simulink model "robot_ver2_testbench"  (R2024b)
settings: Solver=ode4  StartTime=0.0  StopTime=8  FixedStep=0.00050000000000000001  RelTol=1e-6  AbsTol=1e-8
PostLoadFcn:
  | addpath(fileparts(get_param(bdroot,'FileName')), fullfile(fileparts(get_param(bdroot,'FileName')),'src'), fullfile(fileparts(get_param(bdroot,'FileName')),'control'), fullfile(fileparts(get_param(bdroot,'FileName')),'mechanics','URDF_Assembly_Robot_ver2','meshes'));
InitFcn:
  | addpath(fileparts(get_param(bdroot,'FileName')), fullfile(fileparts(get_param(bdroot,'FileName')),'src'), fullfile(fileparts(get_param(bdroot,'FileName')),'control'), fullfile(fileparts(get_param(bdroot,'FileName')),'mechanics','URDF_Assembly_Robot_ver2','meshes'));
model workspace (MAT data in the model file):
  A6 = [0.980198019802; 0.980198019802; 0.980198019802; 0.980198019802; 0.980198019802; 0.980198019802]
  B6 = [0.00049504950495; 0.00049504950495; 0.00049504950495; 0.0049504950495; 0.0049504950495; 0.0049504950495]
  aButter = [1 -1.8226949252 0.837181651256]
  alpha = 0.118088621702
  bButter = [0.00362168151493 0.00724336302986 0.00362168151493]
  bias_est = [0; 0; 0; 0; 0; 0]
  cfg.robotID = 'robot_ver2'
  cfg.mode = 'demonstration'
  cfg.controller = 'c_sil'
  cfg.sampleTime_s = 0.002
  cfg.duration_s = 8
  cfg.gravity_m_s2 = [0 0 -9.81]
  cfg.home_deg = [0 0 -120 60 131.25 0]
  cfg.home_rad = [0 0 -2.09439510239 1.0471975512 2.29074464324 0]
  cfg.provisionalLimits_rad = [-3.14159265359  3.14159265359; -3.14159265359  3.14159265359; -3.14159265359  3.14159265359; -3.14159265359  3.14159265359; -3.14159265359  3.14159265359; -3.14159265359  3.14159265359]
  cfg.minimumLinearInverseCondition = 0.2
  cfg.minimumSelfClearance_m = 0.01
  cfg.minimumEnvironmentClearance_m = 0.01
  cfg.motionCheckStep_rad = 0.00872664625997
  cfg.startupTimeout_s = 15
  cfg.adapter.commandPort = 5006
  cfg.adapter.feedbackPort = 5007
  cfg.adapter.peer = '127.0.0.1'
  cfg.adapter.staleTimeout_s = 0.15
  cfg.adapter.maxJointStep_rad = 0.0349065850399
  cfg.upstream.controlCommit = '15aa22efc071554fe06f1e42e1007633dee15cc9'
  cfg.upstream.admittanceCommit = '589df87e0b36dfb707394ef959a6441456e408e6'
  cfg.demo.status = 'SYNTHETIC_NOT_HARDWARE'
  cfg.demo.reduction = [50 50 50 50 50 50]
  cfg.demo.encoderUnitsPerMotorRev = [32768 32768 32768 32768 32768 32768]
  cfg.demo.direction = [1 1 1 1 1 1]
  cfg.demo.zeroOffset_units = [0 0 0 0 0 0]
  cfg.demo.kp_joint_Nm_rad = [80 120 80 8 5 2]
  cfg.demo.kd_joint_Nm_s_rad = [15 20 12 0.8 0.5 0.2]
  cfg.demo.motorTorqueLimit_Nm = [4 5 4 1 0.8 0.5]
  cfg.demo.motorTorqueTimeConstant_s = 0.002
  cfg.demo.gearEfficiency = [0.9 0.9 0.9 0.9 0.9 0.9]
  cfg.demo.viscousFriction_Nm_s_rad = [0.1 0.1 0.1 0.02 0.02 0.01]
  cfg.demo.jointSpeedLimit_rad_s = [2 2 2 2 2 2]
  cfg.demo.sensor_T_flange = [1  0  0  0; 0  1  0  0; 0  0  1  0; 0  0  0  1]
  cfg.demo.virtualMass = [2 2 2 0.2 0.2 0.2]
  cfg.demo.virtualDamping = [20 20 20 2 2 2]
  cfg.demo.operatorWrench_base_tcp = [1 0 0 0 0 0]
  cfg.demo.wrenchActive_s = [1 3]
  cfg.demo.admittanceSpeedLimit = [0.05 0.05 0.05 0.15 0.15 0.15]
  cfg.demo.admittanceAccelerationLimit = [0.2 0.2 0.2 0.5 0.5 0.5]
  cfg.demo.fullJacobianMinimumSigma = 1e-06
  cfg.hardware.joints(1).motorModel = ''
  cfg.hardware.joints(1).driveModel = ''
  cfg.hardware.joints(1).gearboxModel = ''
  cfg.hardware.joints(1).ratedMotorTorque_Nm = NaN
  cfg.hardware.joints(1).peakMotorTorque_Nm = NaN
  cfg.hardware.joints(1).ratedMotorSpeed_rad_s = NaN
  cfg.hardware.joints(1).maxMotorSpeed_rad_s = NaN
  cfg.hardware.joints(1).ratedCurrent_A = NaN
  cfg.hardware.joints(1).peakCurrent_A = NaN
  cfg.hardware.joints(1).torqueConstant_Nm_A = NaN
  cfg.hardware.joints(1).resistance_Ohm = NaN
  cfg.hardware.joints(1).inductance_H = NaN
  cfg.hardware.joints(1).rotorInertia_kg_m2 = NaN
  cfg.hardware.joints(1).reduction = NaN
  cfg.hardware.joints(1).additionalReduction = NaN
  cfg.hardware.joints(1).gearEfficiency = NaN
  cfg.hardware.joints(1).gearOutputTorqueLimit_Nm = NaN
  cfg.hardware.joints(1).backlash_rad = NaN
  cfg.hardware.joints(1).torsionalStiffness_Nm_rad = NaN
  cfg.hardware.joints(1).encoderUnitsPerMotorRev = NaN
  cfg.hardware.joints(1).direction = NaN
  cfg.hardware.joints(1).zeroOffset_units = NaN
  cfg.hardware.joints(1).positionLimits_rad = [NaN NaN]
  cfg.hardware.joints(1).speedLimit_rad_s = NaN
  cfg.hardware.joints(1).accelerationLimit_rad_s2 = NaN
  cfg.hardware.joints(1).brakePresent = []
  cfg.hardware.joints(1).brakeHoldingTorque_Nm = NaN
  cfg.hardware.joints(1).brakeEngagementTime_s = NaN
  cfg.hardware.joints(1).stopBehavior = ''
  cfg.hardware.joints(1).driveControlParameters = []
  cfg.hardware.joints(1).source = ''
  cfg.hardware.joints(1).verified = 0
  cfg.hardware.joints(2).motorModel = ''
  cfg.hardware.joints(2).driveModel = ''
  cfg.hardware.joints(2).gearboxModel = ''
  cfg.hardware.joints(2).ratedMotorTorque_Nm = NaN
  cfg.hardware.joints(2).peakMotorTorque_Nm = NaN
  cfg.hardware.joints(2).ratedMotorSpeed_rad_s = NaN
  cfg.hardware.joints(2).maxMotorSpeed_rad_s = NaN
  cfg.hardware.joints(2).ratedCurrent_A = NaN
  cfg.hardware.joints(2).peakCurrent_A = NaN
  cfg.hardware.joints(2).torqueConstant_Nm_A = NaN
  cfg.hardware.joints(2).resistance_Ohm = NaN
  cfg.hardware.joints(2).inductance_H = NaN
  cfg.hardware.joints(2).rotorInertia_kg_m2 = NaN
  cfg.hardware.joints(2).reduction = NaN
  cfg.hardware.joints(2).additionalReduction = NaN
  cfg.hardware.joints(2).gearEfficiency = NaN
  cfg.hardware.joints(2).gearOutputTorqueLimit_Nm = NaN
  cfg.hardware.joints(2).backlash_rad = NaN
  cfg.hardware.joints(2).torsionalStiffness_Nm_rad = NaN
  cfg.hardware.joints(2).encoderUnitsPerMotorRev = NaN
  cfg.hardware.joints(2).direction = NaN
  cfg.hardware.joints(2).zeroOffset_units = NaN
  cfg.hardware.joints(2).positionLimits_rad = [NaN NaN]
  cfg.hardware.joints(2).speedLimit_rad_s = NaN
  cfg.hardware.joints(2).accelerationLimit_rad_s2 = NaN
  cfg.hardware.joints(2).brakePresent = []
  cfg.hardware.joints(2).brakeHoldingTorque_Nm = NaN
  cfg.hardware.joints(2).brakeEngagementTime_s = NaN
  cfg.hardware.joints(2).stopBehavior = ''
  cfg.hardware.joints(2).driveControlParameters = []
  cfg.hardware.joints(2).source = ''
  cfg.hardware.joints(2).verified = 0
  cfg.hardware.joints(3).motorModel = ''
  cfg.hardware.joints(3).driveModel = ''
  cfg.hardware.joints(3).gearboxModel = ''
  cfg.hardware.joints(3).ratedMotorTorque_Nm = NaN
  cfg.hardware.joints(3).peakMotorTorque_Nm = NaN
  cfg.hardware.joints(3).ratedMotorSpeed_rad_s = NaN
  cfg.hardware.joints(3).maxMotorSpeed_rad_s = NaN
  cfg.hardware.joints(3).ratedCurrent_A = NaN
  cfg.hardware.joints(3).peakCurrent_A = NaN
  cfg.hardware.joints(3).torqueConstant_Nm_A = NaN
  cfg.hardware.joints(3).resistance_Ohm = NaN
  cfg.hardware.joints(3).inductance_H = NaN
  cfg.hardware.joints(3).rotorInertia_kg_m2 = NaN
  cfg.hardware.joints(3).reduction = NaN
  cfg.hardware.joints(3).additionalReduction = NaN
  cfg.hardware.joints(3).gearEfficiency = NaN
  cfg.hardware.joints(3).gearOutputTorqueLimit_Nm = NaN
  cfg.hardware.joints(3).backlash_rad = NaN
  cfg.hardware.joints(3).torsionalStiffness_Nm_rad = NaN
  cfg.hardware.joints(3).encoderUnitsPerMotorRev = NaN
  cfg.hardware.joints(3).direction = NaN
  cfg.hardware.joints(3).zeroOffset_units = NaN
  cfg.hardware.joints(3).positionLimits_rad = [NaN NaN]
  cfg.hardware.joints(3).speedLimit_rad_s = NaN
  cfg.hardware.joints(3).accelerationLimit_rad_s2 = NaN
  cfg.hardware.joints(3).brakePresent = []
  cfg.hardware.joints(3).brakeHoldingTorque_Nm = NaN
  cfg.hardware.joints(3).brakeEngagementTime_s = NaN
  cfg.hardware.joints(3).stopBehavior = ''
  cfg.hardware.joints(3).driveControlParameters = []
  cfg.hardware.joints(3).source = ''
  cfg.hardware.joints(3).verified = 0
  cfg.hardware.joints(4).motorModel = ''
  cfg.hardware.joints(4).driveModel = ''
  cfg.hardware.joints(4).gearboxModel = ''
  cfg.hardware.joints(4).ratedMotorTorque_Nm = NaN
  cfg.hardware.joints(4).peakMotorTorque_Nm = NaN
  cfg.hardware.joints(4).ratedMotorSpeed_rad_s = NaN
  cfg.hardware.joints(4).maxMotorSpeed_rad_s = NaN
  cfg.hardware.joints(4).ratedCurrent_A = NaN
  cfg.hardware.joints(4).peakCurrent_A = NaN
  cfg.hardware.joints(4).torqueConstant_Nm_A = NaN
  cfg.hardware.joints(4).resistance_Ohm = NaN
  cfg.hardware.joints(4).inductance_H = NaN
  cfg.hardware.joints(4).rotorInertia_kg_m2 = NaN
  cfg.hardware.joints(4).reduction = NaN
  cfg.hardware.joints(4).additionalReduction = NaN
  cfg.hardware.joints(4).gearEfficiency = NaN
  cfg.hardware.joints(4).gearOutputTorqueLimit_Nm = NaN
  cfg.hardware.joints(4).backlash_rad = NaN
  cfg.hardware.joints(4).torsionalStiffness_Nm_rad = NaN
  cfg.hardware.joints(4).encoderUnitsPerMotorRev = NaN
  cfg.hardware.joints(4).direction = NaN
  cfg.hardware.joints(4).zeroOffset_units = NaN
  cfg.hardware.joints(4).positionLimits_rad = [NaN NaN]
  cfg.hardware.joints(4).speedLimit_rad_s = NaN
  cfg.hardware.joints(4).accelerationLimit_rad_s2 = NaN
  cfg.hardware.joints(4).brakePresent = []
  cfg.hardware.joints(4).brakeHoldingTorque_Nm = NaN
  cfg.hardware.joints(4).brakeEngagementTime_s = NaN
  cfg.hardware.joints(4).stopBehavior = ''
  cfg.hardware.joints(4).driveControlParameters = []
  cfg.hardware.joints(4).source = ''
  cfg.hardware.joints(4).verified = 0
  cfg.hardware.joints(5).motorModel = ''
  cfg.hardware.joints(5).driveModel = ''
  cfg.hardware.joints(5).gearboxModel = ''
  cfg.hardware.joints(5).ratedMotorTorque_Nm = NaN
  cfg.hardware.joints(5).peakMotorTorque_Nm = NaN
  cfg.hardware.joints(5).ratedMotorSpeed_rad_s = NaN
  cfg.hardware.joints(5).maxMotorSpeed_rad_s = NaN
  cfg.hardware.joints(5).ratedCurrent_A = NaN
  cfg.hardware.joints(5).peakCurrent_A = NaN
  cfg.hardware.joints(5).torqueConstant_Nm_A = NaN
  cfg.hardware.joints(5).resistance_Ohm = NaN
  cfg.hardware.joints(5).inductance_H = NaN
  cfg.hardware.joints(5).rotorInertia_kg_m2 = NaN
  cfg.hardware.joints(5).reduction = NaN
  cfg.hardware.joints(5).additionalReduction = NaN
  cfg.hardware.joints(5).gearEfficiency = NaN
  cfg.hardware.joints(5).gearOutputTorqueLimit_Nm = NaN
  cfg.hardware.joints(5).backlash_rad = NaN
  cfg.hardware.joints(5).torsionalStiffness_Nm_rad = NaN
  cfg.hardware.joints(5).encoderUnitsPerMotorRev = NaN
  cfg.hardware.joints(5).direction = NaN
  cfg.hardware.joints(5).zeroOffset_units = NaN
  cfg.hardware.joints(5).positionLimits_rad = [NaN NaN]
  cfg.hardware.joints(5).speedLimit_rad_s = NaN
  cfg.hardware.joints(5).accelerationLimit_rad_s2 = NaN
  cfg.hardware.joints(5).brakePresent = []
  cfg.hardware.joints(5).brakeHoldingTorque_Nm = NaN
  cfg.hardware.joints(5).brakeEngagementTime_s = NaN
  cfg.hardware.joints(5).stopBehavior = ''
  cfg.hardware.joints(5).driveControlParameters = []
  cfg.hardware.joints(5).source = ''
  cfg.hardware.joints(5).verified = 0
  cfg.hardware.joints(6).motorModel = ''
  cfg.hardware.joints(6).driveModel = ''
  cfg.hardware.joints(6).gearboxModel = ''
  cfg.hardware.joints(6).ratedMotorTorque_Nm = NaN
  cfg.hardware.joints(6).peakMotorTorque_Nm = NaN
  cfg.hardware.joints(6).ratedMotorSpeed_rad_s = NaN
  cfg.hardware.joints(6).maxMotorSpeed_rad_s = NaN
  cfg.hardware.joints(6).ratedCurrent_A = NaN
  cfg.hardware.joints(6).peakCurrent_A = NaN
  cfg.hardware.joints(6).torqueConstant_Nm_A = NaN
  cfg.hardware.joints(6).resistance_Ohm = NaN
  cfg.hardware.joints(6).inductance_H = NaN
  cfg.hardware.joints(6).rotorInertia_kg_m2 = NaN
  cfg.hardware.joints(6).reduction = NaN
  cfg.hardware.joints(6).additionalReduction = NaN
  cfg.hardware.joints(6).gearEfficiency = NaN
  cfg.hardware.joints(6).gearOutputTorqueLimit_Nm = NaN
  cfg.hardware.joints(6).backlash_rad = NaN
  cfg.hardware.joints(6).torsionalStiffness_Nm_rad = NaN
  cfg.hardware.joints(6).encoderUnitsPerMotorRev = NaN
  cfg.hardware.joints(6).direction = NaN
  cfg.hardware.joints(6).zeroOffset_units = NaN
  cfg.hardware.joints(6).positionLimits_rad = [NaN NaN]
  cfg.hardware.joints(6).speedLimit_rad_s = NaN
  cfg.hardware.joints(6).accelerationLimit_rad_s2 = NaN
  cfg.hardware.joints(6).brakePresent = []
  cfg.hardware.joints(6).brakeHoldingTorque_Nm = NaN
  cfg.hardware.joints(6).brakeEngagementTime_s = NaN
  cfg.hardware.joints(6).stopBehavior = ''
  cfg.hardware.joints(6).driveControlParameters = []
  cfg.hardware.joints(6).source = ''
  cfg.hardware.joints(6).verified = 0
  cfg.hardware.sensor.model = ''
  cfg.hardware.sensor.flange_T_sensor = [NaN  NaN  NaN  NaN; NaN  NaN  NaN  NaN; NaN  NaN  NaN  NaN; NaN  NaN  NaN  NaN]
  cfg.hardware.sensor.sensor_T_grip = [NaN  NaN  NaN  NaN; NaN  NaN  NaN  NaN; NaN  NaN  NaN  NaN; NaN  NaN  NaN  NaN]
  cfg.hardware.sensor.noiseStd = [NaN NaN NaN NaN NaN NaN]
  cfg.hardware.sensor.range = [NaN NaN NaN NaN NaN NaN]
  cfg.hardware.sensor.latency_s = NaN
  cfg.hardware.sensor.protocol = ''
  cfg.hardware.sensor.massAlreadyInCAD = []
  cfg.hardware.sensor.verified = 0
  cfg.hardware.actuatorModelValidated = 0
  cfg.hardware.massAccountingVerified = 0
  cfg.hardware.stopBehaviorValidated = 0
  cfg.hardware.source = ''
  cfg.environment(1).name = 'Floor'
  cfg.environment(1).size_m = [3 3 0.05]
  cfg.environment(1).center_m = [0 0 -0.08]
  cfg.environment(1).rpy_rad = [0 0 0]
  cfg.environment(2).name = 'Workpiece'
  cfg.environment(2).size_m = [0.3 0.3 0.1]
  cfg.environment(2).center_m = [0.85 0.65 0.35]
  cfg.environment(2).rpy_rad = [0 0 0]
  cfg.sensor.bias = [0; 0; 0; 0; 0; 0]
  cfg.sensor.noise_std = [0.08; 0.08; 0.06; 0.004; 0.004; 0.003]
  cfg.sensor.drift_per_s = [0.005; 0.003; -0.004; 0.0002; 0; 0]
  cfg.sensor.coupling = [1  0  0  0  0  0; 0  1  0  0  0  0; 0  0  1  0  0  0; 0  0  0  1  0  0; 0  0  0  0  1  0; 0  0  0  0  0  1]
  cfg.sensor.quantization_step = [0.01; 0.01; 0.01; 0.001; 0.001; 0.001]
  cfg.sensor.saturation = [100; 100; 100; 10; 10; 10]
  cfg.sensor.filterCutoff_Hz = 10
  cfg.sensor.seed = 17
  configurationSHA256 = '837b8b2e35843bef305e3cf046f537b0ec4730ac609ea7d1386ea74f346316b0'
  initialQ = [0 0 -2.09439510239 1.0471975512 2.29074464324 0]
  packagedUrdfSHA256 = '4375e6be56b72db950ac87d5631842c692121a0d0489fcb89f928996cc18049b'
undefined symbols (not defined in the file or in its folder): X, Y, Z
libraries: sm_lib x68, nesl_utility x29
(part 1 of 2)
settings Model: Creator=pc  LastModifiedBy=pc

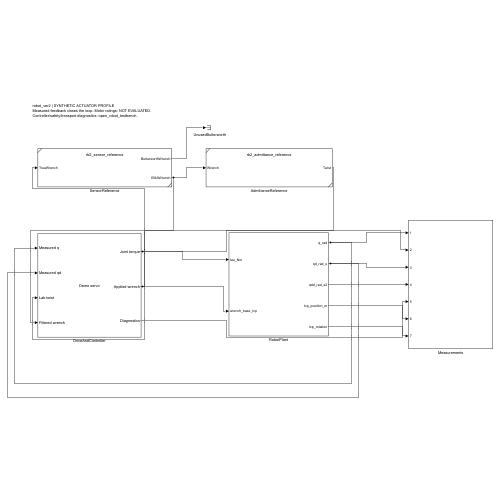
[thumbnail: Simulink's stored preview of the top-level diagram]
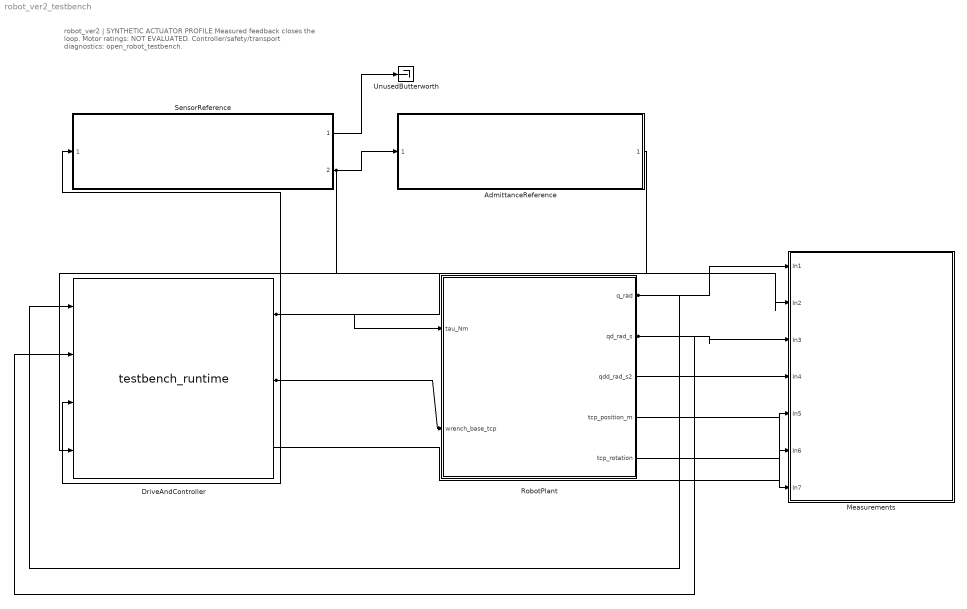
== system robot_ver2_testbench ==
  note: robot_ver2 | SYNTHETIC ACTUATOR PROFILE
      | Measured feedback closes the loop. Motor ratings: NOT EVALUATED.
      | Controller/safety/transport diagnostics: open_robot_testbench.
  AdmittanceReference : Subsystem  ReferencedSubsystem=rb2_admittance_reference
  DriveAndController : M-S-Function  FunctionName=testbench_runtime
      mask Display:
      | disp('Demo servo');
      | port_label('input',1,'Measured q');port_label('input',2,'Measured qd');
      | port_label('input',3,'Lab twist');port_label('input',4,'Filtered wrench');
      | port_label('output',1,'Joint torque');port_label('output',2,'Applied wrench');
      | port_label('output',3,'Diagnostics');
  Measurements : Subsystem
  RobotPlant : Subsystem
  SensorReference : Subsystem  ReferencedSubsystem=rb2_sensor_reference
  UnusedButterworth : Terminator
  wires:
  SensorReference/2 -> AdmittanceReference/1, DriveAndController/4
  RobotPlant/1(q_rad) -> DriveAndController/1, Measurements/1(In1)
  RobotPlant/2(qd_rad_s) -> DriveAndController/2, Measurements/3(In3)
  AdmittanceReference/1 -> DriveAndController/3
  DriveAndController/1 -> Measurements/2(In2), RobotPlant/1(tau_Nm)
  RobotPlant/3(qdd_rad_s2) -> Measurements/4(In4)
  DriveAndController/3 -> Measurements/5(In5)
  RobotPlant/4(tcp_position_m) -> Measurements/6(In6)
  RobotPlant/5(tcp_rotation) -> Measurements/7(In7)
  DriveAndController/2 -> RobotPlant/2(wrench_base_tcp), SensorReference/1
  SensorReference/1 -> UnusedButterworth/1

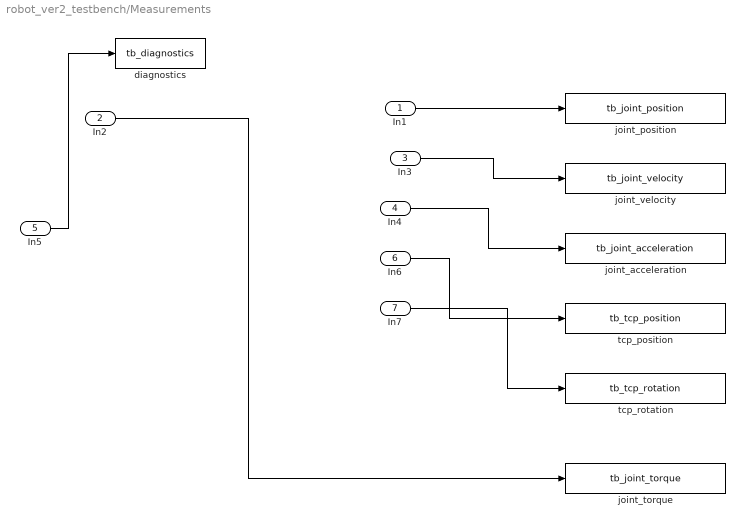
== system robot_ver2_testbench/Measurements ==
  In1 : Inport
  In2 : Inport  Port=2
  In3 : Inport  Port=3
  In4 : Inport  Port=4
  In5 : Inport  Port=5
  In6 : Inport  Port=6
  In7 : Inport  Port=7
  diagnostics : ToWorkspace  VariableName=tb_diagnostics  SaveFormat=Timeseries  SampleTime=-1
  joint_acceleration : ToWorkspace  VariableName=tb_joint_acceleration  SaveFormat=Timeseries  SampleTime=-1
  joint_position : ToWorkspace  VariableName=tb_joint_position  SaveFormat=Timeseries  SampleTime=-1
  joint_torque : ToWorkspace  VariableName=tb_joint_torque  SaveFormat=Timeseries  SampleTime=-1
  joint_velocity : ToWorkspace  VariableName=tb_joint_velocity  SaveFormat=Timeseries  SampleTime=-1
  tcp_position : ToWorkspace  VariableName=tb_tcp_position  SaveFormat=Timeseries  SampleTime=-1
  tcp_rotation : ToWorkspace  VariableName=tb_tcp_rotation  SaveFormat=Timeseries  SampleTime=-1
  wires:
  In7/1 -> tcp_rotation/1
  In3/1 -> joint_velocity/1
  In5/1 -> diagnostics/1
  In6/1 -> tcp_position/1
  In2/1 -> joint_torque/1
  In4/1 -> joint_acceleration/1
  In1/1 -> joint_position/1

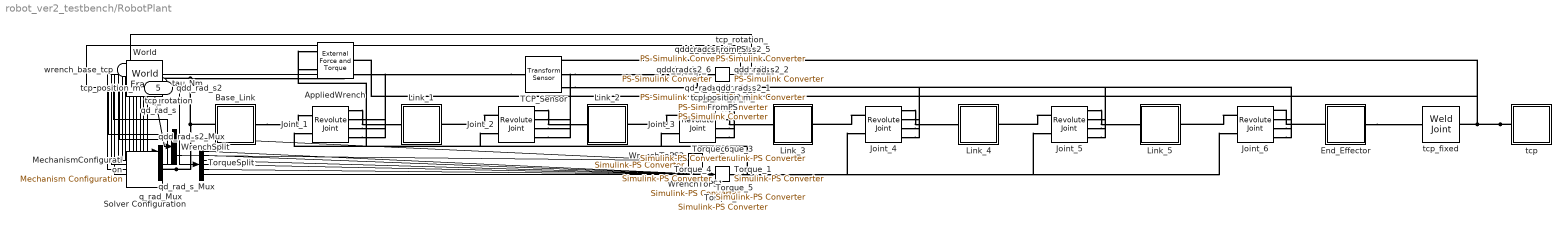
== system robot_ver2_testbench/RobotPlant ==
  tau_Nm : Inport  PortDimensions=6
  wrench_base_tcp : Inport  Port=2  PortDimensions=6
  AppliedWrench : sm_lib/Forces and Torques/External Force and Torque  EnableForceX=off  EnableForceY=off  EnableForceZ=off  EnableForce=on  ForceResolutionFrame=World  EnableTorqueX=off  EnableTorqueY=off  EnableTorqueZ=off  EnableTorque=on  TorqueResolutionFrame=World
  Base_Link : Subsystem
  End_Effector : Subsystem
  Joint_1 : sm_lib/Joints/Revolute Joint  JointMode=Normal  CompositeWrenchDir=FollowerOnBase  CompositeWrenchFrame=BaseFrame  SenseConstraintForce=off  SenseConstraintTorque=off  SenseTotalForce=off  SenseTotalTorque=off  PositionTargetSpecify=on  PositionTargetPriority=High  PositionTargetValue=initialQ(1)  PositionTargetValueUnits=rad  VelocityTargetSpecify=on  VelocityTargetPriority=High  VelocityTargetValue=0  VelocityTargetValueUnits=rad/s  EquilibriumPosition=0  EquilibriumPositionUnits=deg  SpringStiffness=0  SpringStiffnessUnits=N*m/deg  DampingCoefficient=0  DampingCoefficientUnits=kg*m^2/(rad*s)  LowerLimitSpecify=on  LowerLimitBound=-3.141592653589793  LowerLimitBoundUnits=rad  LowerLimitStiffness=1e4  LowerLimitStiffnessUnits=N*m/deg  LowerLimitDamping=10  LowerLimitDampingUnits=N*m/(deg/s)  LowerLimitTransitionRegionWidth=0.1  LowerLimitTransitionRegionWidthUnits=deg  UpperLimitSpecify=on  UpperLimitBound=3.141592653589793  UpperLimitBoundUnits=rad  UpperLimitStiffness=1e4  UpperLimitStiffnessUnits=N*m/deg  UpperLimitDamping=10  UpperLimitDampingUnits=N*m/(deg/s)  UpperLimitTransitionRegionWidth=0.1  UpperLimitTransitionRegionWidthUnits=deg  TorqueActuationMode=InputTorque  MotionActuationMode=ComputedMotion  SensePosition=on  SenseVelocity=on  SenseAcceleration=on  SenseTorqueForce=off  SenseLowerLimitTorqueForce=off  SenseUpperLimitTorqueForce=off
  Joint_2 : sm_lib/Joints/Revolute Joint  JointMode=Normal  CompositeWrenchDir=FollowerOnBase  CompositeWrenchFrame=BaseFrame  SenseConstraintForce=off  SenseConstraintTorque=off  SenseTotalForce=off  SenseTotalTorque=off  PositionTargetSpecify=on  PositionTargetPriority=High  PositionTargetValue=initialQ(2)  PositionTargetValueUnits=rad  VelocityTargetSpecify=on  VelocityTargetPriority=High  VelocityTargetValue=0  VelocityTargetValueUnits=rad/s  EquilibriumPosition=0  EquilibriumPositionUnits=deg  SpringStiffness=0  SpringStiffnessUnits=N*m/deg  DampingCoefficient=0  DampingCoefficientUnits=kg*m^2/(rad*s)  LowerLimitSpecify=on  LowerLimitBound=-3.141592653589793  LowerLimitBoundUnits=rad  LowerLimitStiffness=1e4  LowerLimitStiffnessUnits=N*m/deg  LowerLimitDamping=10  LowerLimitDampingUnits=N*m/(deg/s)  LowerLimitTransitionRegionWidth=0.1  LowerLimitTransitionRegionWidthUnits=deg  UpperLimitSpecify=on  UpperLimitBound=3.141592653589793  UpperLimitBoundUnits=rad  UpperLimitStiffness=1e4  UpperLimitStiffnessUnits=N*m/deg  UpperLimitDamping=10  UpperLimitDampingUnits=N*m/(deg/s)  UpperLimitTransitionRegionWidth=0.1  UpperLimitTransitionRegionWidthUnits=deg  TorqueActuationMode=InputTorque  MotionActuationMode=ComputedMotion  SensePosition=on  SenseVelocity=on  SenseAcceleration=on  SenseTorqueForce=off  SenseLowerLimitTorqueForce=off  SenseUpperLimitTorqueForce=off
  Joint_3 : sm_lib/Joints/Revolute Joint  JointMode=Normal  CompositeWrenchDir=FollowerOnBase  CompositeWrenchFrame=BaseFrame  SenseConstraintForce=off  SenseConstraintTorque=off  SenseTotalForce=off  SenseTotalTorque=off  PositionTargetSpecify=on  PositionTargetPriority=High  PositionTargetValue=initialQ(3)  PositionTargetValueUnits=rad  VelocityTargetSpecify=on  VelocityTargetPriority=High  VelocityTargetValue=0  VelocityTargetValueUnits=rad/s  EquilibriumPosition=0  EquilibriumPositionUnits=deg  SpringStiffness=0  SpringStiffnessUnits=N*m/deg  DampingCoefficient=0  DampingCoefficientUnits=kg*m^2/(rad*s)  LowerLimitSpecify=on  LowerLimitBound=-3.141592653589793  LowerLimitBoundUnits=rad  LowerLimitStiffness=1e4  LowerLimitStiffnessUnits=N*m/deg  LowerLimitDamping=10  LowerLimitDampingUnits=N*m/(deg/s)  LowerLimitTransitionRegionWidth=0.1  LowerLimitTransitionRegionWidthUnits=deg  UpperLimitSpecify=on  UpperLimitBound=3.141592653589793  UpperLimitBoundUnits=rad  UpperLimitStiffness=1e4  UpperLimitStiffnessUnits=N*m/deg  UpperLimitDamping=10  UpperLimitDampingUnits=N*m/(deg/s)  UpperLimitTransitionRegionWidth=0.1  UpperLimitTransitionRegionWidthUnits=deg  TorqueActuationMode=InputTorque  MotionActuationMode=ComputedMotion  SensePosition=on  SenseVelocity=on  SenseAcceleration=on  SenseTorqueForce=off  SenseLowerLimitTorqueForce=off  SenseUpperLimitTorqueForce=off
  Joint_4 : sm_lib/Joints/Revolute Joint  JointMode=Normal  CompositeWrenchDir=FollowerOnBase  CompositeWrenchFrame=BaseFrame  SenseConstraintForce=off  SenseConstraintTorque=off  SenseTotalForce=off  SenseTotalTorque=off  PositionTargetSpecify=on  PositionTargetPriority=High  PositionTargetValue=initialQ(4)  PositionTargetValueUnits=rad  VelocityTargetSpecify=on  VelocityTargetPriority=High  VelocityTargetValue=0  VelocityTargetValueUnits=rad/s  EquilibriumPosition=0  EquilibriumPositionUnits=deg  SpringStiffness=0  SpringStiffnessUnits=N*m/deg  DampingCoefficient=0  DampingCoefficientUnits=kg*m^2/(rad*s)  LowerLimitSpecify=on  LowerLimitBound=-3.141592653589793  LowerLimitBoundUnits=rad  LowerLimitStiffness=1e4  LowerLimitStiffnessUnits=N*m/deg  LowerLimitDamping=10  LowerLimitDampingUnits=N*m/(deg/s)  LowerLimitTransitionRegionWidth=0.1  LowerLimitTransitionRegionWidthUnits=deg  UpperLimitSpecify=on  UpperLimitBound=3.141592653589793  UpperLimitBoundUnits=rad  UpperLimitStiffness=1e4  UpperLimitStiffnessUnits=N*m/deg  UpperLimitDamping=10  UpperLimitDampingUnits=N*m/(deg/s)  UpperLimitTransitionRegionWidth=0.1  UpperLimitTransitionRegionWidthUnits=deg  TorqueActuationMode=InputTorque  MotionActuationMode=ComputedMotion  SensePosition=on  SenseVelocity=on  SenseAcceleration=on  SenseTorqueForce=off  SenseLowerLimitTorqueForce=off  SenseUpperLimitTorqueForce=off
  Joint_5 : sm_lib/Joints/Revolute Joint  JointMode=Normal  CompositeWrenchDir=FollowerOnBase  CompositeWrenchFrame=BaseFrame  SenseConstraintForce=off  SenseConstraintTorque=off  SenseTotalForce=off  SenseTotalTorque=off  PositionTargetSpecify=on  PositionTargetPriority=High  PositionTargetValue=initialQ(5)  PositionTargetValueUnits=rad  VelocityTargetSpecify=on  VelocityTargetPriority=High  VelocityTargetValue=0  VelocityTargetValueUnits=rad/s  EquilibriumPosition=0  EquilibriumPositionUnits=deg  SpringStiffness=0  SpringStiffnessUnits=N*m/deg  DampingCoefficient=0  DampingCoefficientUnits=kg*m^2/(rad*s)  LowerLimitSpecify=on  LowerLimitBound=-3.141592653589793  LowerLimitBoundUnits=rad  LowerLimitStiffness=1e4  LowerLimitStiffnessUnits=N*m/deg  LowerLimitDamping=10  LowerLimitDampingUnits=N*m/(deg/s)  LowerLimitTransitionRegionWidth=0.1  LowerLimitTransitionRegionWidthUnits=deg  UpperLimitSpecify=on  UpperLimitBound=3.141592653589793  UpperLimitBoundUnits=rad  UpperLimitStiffness=1e4  UpperLimitStiffnessUnits=N*m/deg  UpperLimitDamping=10  UpperLimitDampingUnits=N*m/(deg/s)  UpperLimitTransitionRegionWidth=0.1  UpperLimitTransitionRegionWidthUnits=deg  TorqueActuationMode=InputTorque  MotionActuationMode=ComputedMotion  SensePosition=on  SenseVelocity=on  SenseAcceleration=on  SenseTorqueForce=off  SenseLowerLimitTorqueForce=off  SenseUpperLimitTorqueForce=off
  Joint_6 : sm_lib/Joints/Revolute Joint  JointMode=Normal  CompositeWrenchDir=FollowerOnBase  CompositeWrenchFrame=BaseFrame  SenseConstraintForce=off  SenseConstraintTorque=off  SenseTotalForce=off  SenseTotalTorque=off  PositionTargetSpecify=on  PositionTargetPriority=High  PositionTargetValue=initialQ(6)  PositionTargetValueUnits=rad  VelocityTargetSpecify=on  VelocityTargetPriority=High  VelocityTargetValue=0  VelocityTargetValueUnits=rad/s  EquilibriumPosition=0  EquilibriumPositionUnits=deg  SpringStiffness=0  SpringStiffnessUnits=N*m/deg  DampingCoefficient=0  DampingCoefficientUnits=kg*m^2/(rad*s)  LowerLimitSpecify=on  LowerLimitBound=-3.141592653589793  LowerLimitBoundUnits=rad  LowerLimitStiffness=1e4  LowerLimitStiffnessUnits=N*m/deg  LowerLimitDamping=10  LowerLimitDampingUnits=N*m/(deg/s)  LowerLimitTransitionRegionWidth=0.1  LowerLimitTransitionRegionWidthUnits=deg  UpperLimitSpecify=on  UpperLimitBound=3.141592653589793  UpperLimitBoundUnits=rad  UpperLimitStiffness=1e4  UpperLimitStiffnessUnits=N*m/deg  UpperLimitDamping=10  UpperLimitDampingUnits=N*m/(deg/s)  UpperLimitTransitionRegionWidth=0.1  UpperLimitTransitionRegionWidthUnits=deg  TorqueActuationMode=InputTorque  MotionActuationMode=ComputedMotion  SensePosition=on  SenseVelocity=on  SenseAcceleration=on  SenseTorqueForce=off  SenseLowerLimitTorqueForce=off  SenseUpperLimitTorqueForce=off
  Link_1 : Subsystem
  Link_2 : Subsystem
  Link_3 : Subsystem
  Link_4 : Subsystem
  Link_5 : Subsystem
  MechanismConfiguration : sm_lib/Utilities/Mechanism Configuration  UniformGravity=Constant  GravityVector=[0 0 -9.8100000000000005]  GravityVectorUnits=m/s^2  LinearizationDelta=0.001  JointModeTransitionNonlinearIterations=2
  Solver Configuration : nesl_utility/Solver Configuration  PhysicalDomain=network_engine_domain  SubClassName=solver  LeftPortType=input  RightPortType=generic  Tones=[]  Harmonics=[]  SimulateNoise=off  Profile=off  UseLocalSampling=off  EnableSwitchedLinearOptims=on  FrequencyDomain=off  UseCCode=off  RelTol=0.001  AbsTol=0.001  MinStep=1e-09  ToWorkspace=off  RevertToSquareIcSolve=off  NumHomotopyIterations=100  PhasorMode=off  PhasorModeNumHarmonics=1  ConsistencySolver=NEWTON_XTOL_AFTER_FTOL  IndexReductionMethod=DerivativeReplacement  DoDC=off  ResidualTolerance=1e-09  ConsistencyTolSource=GLOBAL  ConsistencyAbsTol=0.001  ConsistencyRelTol=0.001  ConsistencyTolFactor=0.001  UseLocalSolver=off  LocalSolverChoice=NE_BACKWARD_EULER_ADVANCER  ResolveIndetEquations=on  FunctionEvalNumThread=1  LocalSolverSampleTime=0.001  DoFixedCost=off  MaxNonlinIter=3  MaxModeIter=2  ComputeImpulses=off  ImpulseIterations=2  LinearAlgebra=auto  LinearAlgebraNumThread=0  EquationFormulation=NE_TIME_EF  DelaysMemoryBudget=1024  AutomaticFiltering=on  FilteringTimeConstant=0.001  PartitionStorageMethod=AS_NEEDED  PartitionMemoryBudget=1024  PartitionMethod=ROBUST  MultibodyUseLocalSolver=off  MultibodyLocalSolverChoice=ODE1  MultibodyLocalSolverSampleTime=0.001
  TCP_Sensor : sm_lib/Frames and Transforms/Transform Sensor  MeasurementFrame=World  RotationSequence=XYX  SenseAngle=off  SenseAxis=off  SenseQ=off  SenseR=on  SenseRotationSequence=off  SenseOmegaX=off  SenseOmegaY=off  SenseOmegaZ=off  SenseOmega=off  SenseQDot=off  SenseRDot=off  SenseRotationSequenceDot=off  SenseAlphaX=off  SenseAlphaY=off  SenseAlphaZ=off  SenseAlpha=off  SenseQDDot=off  SenseRDDot=off  SenseX=off  SenseY=off  SenseZ=off  SenseXYZ=on  SenseRad=off  SenseAzim=off  SenseDist=off  SenseInc=off  SenseXDot=off  SenseYDot=off  SenseZDot=off  SenseXYZDot=off  SenseRadDot=off  SenseAzimDot=off  SenseDistDot=off  SenseIncDot=off  SenseXDDot=off  SenseYDDot=off  SenseZDDot=off  SenseXYZDDot=off  SenseRadDDot=off  SenseAzimDDot=off  SenseDistDDot=off  SenseIncDDot=off
  TorqueSplit : Demux  Outputs=6
  Torque_{1..6} (6 alike) : nesl_utility/Simulink-PS Converter  PhysicalDomain=network_engine_domain  SubClassName=ps_input  LeftPortType=input  RightPortType=output  PseudoPeriodic=off  Frequencies=[]  NoiseDistribution=none  NoiseParameters=[]  Unit=N*m  AffineConversion=off  FilteringAndDerivatives=provide  SimscapeFilterOrder=1  InputFilterTimeConstant=0.001  UdotUserProvided=0
  World : sm_lib/Frames and Transforms/World Frame
  WrenchSplit : Demux  Outputs=[3 3]
  WrenchToPS1 : nesl_utility/Simulink-PS Converter  PhysicalDomain=network_engine_domain  SubClassName=ps_input  LeftPortType=input  RightPortType=output  PseudoPeriodic=off  Frequencies=[]  NoiseDistribution=none  NoiseParameters=[]  Unit=N  AffineConversion=off  FilteringAndDerivatives=provide  SimscapeFilterOrder=1  InputFilterTimeConstant=0.001  UdotUserProvided=0
  WrenchToPS2 : nesl_utility/Simulink-PS Converter  PhysicalDomain=network_engine_domain  SubClassName=ps_input  LeftPortType=input  RightPortType=output  PseudoPeriodic=off  Frequencies=[]  NoiseDistribution=none  NoiseParameters=[]  Unit=N*m  AffineConversion=off  FilteringAndDerivatives=provide  SimscapeFilterOrder=1  InputFilterTimeConstant=0.001  UdotUserProvided=0
  q_rad_{1..6} (6 alike) : nesl_utility/PS-Simulink Converter  PhysicalDomain=network_engine_domain  SubClassName=ps_output  LeftPortType=input  RightPortType=output  PseudoPeriodic=off  Frequencies=[]  VectorFormat=inherit  Unit=rad  AffineConversion=off
  q_rad_Mux : Mux  Inputs=6
  qd_rad_s_{1..6} (6 alike) : nesl_utility/PS-Simulink Converter  PhysicalDomain=network_engine_domain  SubClassName=ps_output  LeftPortType=input  RightPortType=output  PseudoPeriodic=off  Frequencies=[]  VectorFormat=inherit  Unit=rad/s  AffineConversion=off
  qd_rad_s_Mux : Mux  Inputs=6
  qdd_rad_s2_{1..6} (6 alike) : nesl_utility/PS-Simulink Converter  PhysicalDomain=network_engine_domain  SubClassName=ps_output  LeftPortType=input  RightPortType=output  PseudoPeriodic=off  Frequencies=[]  VectorFormat=inherit  Unit=rad/s^2  AffineConversion=off
  qdd_rad_s2_Mux : Mux  Inputs=6
  tcp : Subsystem
  tcp_fixed : sm_lib/Joints/Weld Joint  JointMode=Normal  CompositeWrenchDir=FollowerOnBase  CompositeWrenchFrame=BaseFrame  SenseConstraintForce=off  SenseConstraintTorque=off  SenseTotalForce=off  SenseTotalTorque=off
  tcp_position_m_FromPS : nesl_utility/PS-Simulink Converter  PhysicalDomain=network_engine_domain  SubClassName=ps_output  LeftPortType=input  RightPortType=output  PseudoPeriodic=off  Frequencies=[]  VectorFormat=inherit  Unit=m  AffineConversion=off
  tcp_rotation_FromPS : nesl_utility/PS-Simulink Converter  PhysicalDomain=network_engine_domain  SubClassName=ps_output  LeftPortType=input  RightPortType=output  PseudoPeriodic=off  Frequencies=[]  VectorFormat=inherit  Unit=1  AffineConversion=off
  q_rad : Outport
  qd_rad_s : Outport  Port=2
  qdd_rad_s2 : Outport  Port=3
  tcp_position_m : Outport  Port=4
  tcp_rotation : Outport  Port=5
  wires:
  qdd_rad_s2_2/1 -> qdd_rad_s2_Mux/2
  q_rad_2/1 -> q_rad_Mux/2
  qd_rad_s_2/1 -> qd_rad_s_Mux/2
  TorqueSplit/2 -> Torque_2/1
  qd_rad_s_Mux/1 -> qd_rad_s/1
  TorqueSplit/5 -> Torque_5/1
  qd_rad_s_5/1 -> qd_rad_s_Mux/5
  qdd_rad_s2_6/1 -> qdd_rad_s2_Mux/6
  TorqueSplit/1 -> Torque_1/1
  TorqueSplit/6 -> Torque_6/1
  qdd_rad_s2_4/1 -> qdd_rad_s2_Mux/4
  qdd_rad_s2_3/1 -> qdd_rad_s2_Mux/3
  q_rad_3/1 -> q_rad_Mux/3
  qd_rad_s_4/1 -> qd_rad_s_Mux/4
  q_rad_6/1 -> q_rad_Mux/6
  tcp_position_m_FromPS/1 -> tcp_position_m/1
  qdd_rad_s2_Mux/1 -> qdd_rad_s2/1
  q_rad_4/1 -> q_rad_Mux/4
  qdd_rad_s2_5/1 -> qdd_rad_s2_Mux/5
  qd_rad_s_3/1 -> qd_rad_s_Mux/3
  qd_rad_s_1/1 -> qd_rad_s_Mux/1
  tcp_rotation_FromPS/1 -> tcp_rotation/1
  qdd_rad_s2_1/1 -> qdd_rad_s2_Mux/1
  q_rad_5/1 -> q_rad_Mux/5
  q_rad_Mux/1 -> q_rad/1
  tau_Nm/1 -> TorqueSplit/1
  qd_rad_s_6/1 -> qd_rad_s_Mux/6
  q_rad_1/1 -> q_rad_Mux/1
  TorqueSplit/3 -> Torque_3/1
  TorqueSplit/4 -> Torque_4/1
  wrench_base_tcp/1 -> WrenchSplit/1
  WrenchSplit/1 -> WrenchToPS1/1
  WrenchSplit/2 -> WrenchToPS2/1
  connections:
  Joint_2/RConn2 -- q_rad_2/LConn1
  Torque_2/RConn1 -- Joint_2/LConn2
  Joint_1/RConn4 -- qdd_rad_s2_1/LConn1
  Joint_2/RConn3 -- qd_rad_s_2/LConn1
  Joint_2/RConn4 -- qdd_rad_s2_2/LConn1
  TCP_Sensor/RConn3 -- tcp_position_m_FromPS/LConn1
  Joint_5/RConn3 -- qd_rad_s_5/LConn1
  Torque_1/RConn1 -- Joint_1/LConn2
  Joint_4/RConn2 -- q_rad_4/LConn1
  Joint_3/RConn3 -- qd_rad_s_3/LConn1
  Joint_6/RConn4 -- qdd_rad_s2_6/LConn1
  Joint_3/RConn2 -- q_rad_3/LConn1
  Torque_3/RConn1 -- Joint_3/LConn2
  Joint_4/RConn4 -- qdd_rad_s2_4/LConn1
  Torque_4/RConn1 -- Joint_4/LConn2
  Joint_1/RConn3 -- qd_rad_s_1/LConn1
  Joint_1/RConn1 -- Link_1/LConn1
  Joint_4/RConn3 -- qd_rad_s_4/LConn1
  End_Effector/LConn1 -- Joint_6/RConn1
  Torque_6/RConn1 -- Joint_6/LConn2
  Base_Link/RConn1 -- Joint_1/LConn1
  End_Effector/RConn1 -- tcp_fixed/LConn1
  Joint_3/LConn1 -- Link_2/RConn1
  Joint_5/RConn4 -- qdd_rad_s2_5/LConn1
  Joint_3/RConn1 -- Link_3/LConn1
  Joint_5/RConn2 -- q_rad_5/LConn1
  Joint_2/RConn1 -- Link_2/LConn1
  Torque_5/RConn1 -- Joint_5/LConn2
  Joint_6/RConn3 -- qd_rad_s_6/LConn1
  Joint_4/LConn1 -- Link_3/RConn1
  Joint_4/RConn1 -- Link_4/LConn1
  Joint_5/RConn1 -- Link_5/LConn1
  Joint_5/LConn1 -- Link_4/RConn1
  Joint_1/RConn2 -- q_rad_1/LConn1
  Joint_6/LConn1 -- Link_5/RConn1
  TCP_Sensor/RConn2 -- tcp_rotation_FromPS/LConn1
  Joint_6/RConn2 -- q_rad_6/LConn1
  TCP_Sensor/LConn1 -- World/RConn1 -- Solver Configuration/RConn1 -- MechanismConfiguration/RConn1 -- Base_Link/LConn1
  TCP_Sensor/RConn1 -- tcp/LConn1 -- AppliedWrench/RConn1 -- tcp_fixed/RConn1
  Joint_3/RConn4 -- qdd_rad_s2_3/LConn1
  Joint_2/LConn1 -- Link_1/RConn1
  WrenchToPS1/RConn1 -- AppliedWrench/LConn1
  WrenchToPS2/RConn1 -- AppliedWrench/LConn2

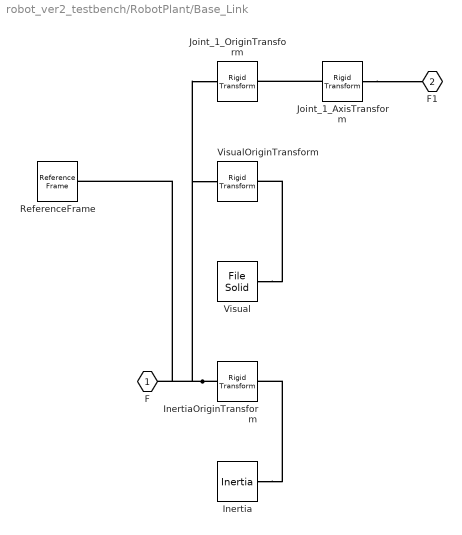
== system robot_ver2_testbench/RobotPlant/Base_Link ==
  Inertia : sm_lib/Body Elements/Inertia  InertiaType=Custom  Mass=4.45952773181733  MassUnits=kg  CenterOfMass=[0, 0, 0]  CenterOfMassUnits=m  MomentsOfInertia=[0.0365014937398595, 0.0365014937398595, 0.0432728026009368]  MomentsOfInertiaUnits=kg*m^2  ProductsOfInertia=[-1.63931612712631e-18, 3.25877544074145e-19, -1.11173074327127e-18]  ProductsOfInertiaUnits=kg*m^2  GraphicType=None  MarkerShape=Inertia  MarkerSize=20  GraphicVisPropType=SimpleVisualProperties  GraphicDiffuseColor=[0.5 0.5 0.5]  GraphicOpacity=1  GraphicSpecularColor=[0.5 0.5 0.5 1.0]  GraphicAmbientColor=[0.15 0.15 0.15 1.0]  GraphicEmissiveColor=[0.0 0.0 0.0 1.0]  GraphicShininess=75
  InertiaOriginTransform : sm_lib/Frames and Transforms/Rigid Transform  RotationMethod=RotationSequence  FollAlignAxisA=+X  BaseAlignAxisA=+Y  FollAlignAxisB=+Y  BaseAlignAxisB=+Z  RotationStandardAxis=+Z  RotationAngle=0  RotationAngleUnits=deg  RotationArbitraryAxis=[0 0 1]  RotationSequenceAxes=BaseAxes  RotationSequence=XYZ  RotationSequenceAngles=[0, 0, 0]  RotationSequenceAnglesUnits=rad  RotationMatrix=[1 0 0;0 1 0;0 0 1]  Quaternion=[1 0 0 0]  TranslationMethod=Cartesian  TranslationCartesianOffset=[7.32447693854411e-18, -1.19067266926414e-17, 0.1]  TranslationCartesianOffsetUnits=m  TranslationStandardAxis=+Z  TranslationStandardOffset=0  TranslationStandardOffsetUnits=m  TranslationROffset=0  TranslationROffsetUnits=m  TranslationThetaOffset=0  TranslationThetaOffsetUnits=deg  TranslationZOffset=0  TranslationZOffsetUnits=m
  Joint_1_AxisTransform : sm_lib/Frames and Transforms/Rigid Transform  RotationMethod=ArbitraryAxis  FollAlignAxisA=+X  BaseAlignAxisA=+Y  FollAlignAxisB=+Y  BaseAlignAxisB=+Z  RotationStandardAxis=+Z  RotationAngle=3.141592653589793  RotationAngleUnits=rad  RotationArbitraryAxis=[1, 0, 0]  RotationSequenceAxes=FollowerAxes  RotationSequence=XYX  RotationSequenceAngles=[0 0 0]  RotationSequenceAnglesUnits=deg  RotationMatrix=[1 0 0;0 1 0;0 0 1]  Quaternion=[1 0 0 0]  TranslationMethod=Cartesian  TranslationCartesianOffset=[0, 0, 0]  TranslationCartesianOffsetUnits=m  TranslationStandardAxis=+Z  TranslationStandardOffset=0  TranslationStandardOffsetUnits=m  TranslationROffset=0  TranslationROffsetUnits=m  TranslationThetaOffset=0  TranslationThetaOffsetUnits=deg  TranslationZOffset=0  TranslationZOffsetUnits=m
  Joint_1_OriginTransform : sm_lib/Frames and Transforms/Rigid Transform  RotationMethod=RotationSequence  FollAlignAxisA=+X  BaseAlignAxisA=+Y  FollAlignAxisB=+Y  BaseAlignAxisB=+Z  RotationStandardAxis=+Z  RotationAngle=0  RotationAngleUnits=deg  RotationArbitraryAxis=[0 0 1]  RotationSequenceAxes=BaseAxes  RotationSequence=XYZ  RotationSequenceAngles=[0, 0, 0]  RotationSequenceAnglesUnits=rad  RotationMatrix=[1 0 0;0 1 0;0 0 1]  Quaternion=[1 0 0 0]  TranslationMethod=Cartesian  TranslationCartesianOffset=[0, 0, 0.2]  TranslationCartesianOffsetUnits=m  TranslationStandardAxis=+Z  TranslationStandardOffset=0  TranslationStandardOffsetUnits=m  TranslationROffset=0  TranslationROffsetUnits=m  TranslationThetaOffset=0  TranslationThetaOffsetUnits=deg  TranslationZOffset=0  TranslationZOffsetUnits=m
  ReferenceFrame : sm_lib/Frames and Transforms/Reference Frame
  Visual : sm_lib/Body Elements/File Solid  ExtGeomFileName=robot_ver2_Base_Link.STL  UnitType=Custom  ExtGeomFileUnits=m  StepReaderType=HEX  ExportConvexHullGeometry=off  InertiaType=Custom  BasedOnType=DensityFromFile  Density=1000  DensityUnits=kg/m^3  Mass=0  MassUnits=kg  CenterOfMass=[0, 0, 0]  CenterOfMassUnits=m  MomentsOfInertia=[0, 0, 0]  MomentsOfInertiaUnits=kg*m^2  ProductsOfInertia=[0, 0, 0]  ProductsOfInertiaUnits=kg*m^2  GraphicType=FromGeometry  MarkerShape=Sphere  MarkerSize=10  GraphicVisPropType=SimpleVisualProperties  GraphicDiffuseColor=[0.792156862745098, 0.819607843137255, 0.933333333333333]  GraphicOpacity=1  GraphicSpecularColor=[0.5 0.5 0.5 1.0]  GraphicAmbientColor=[0.15 0.15 0.15 1.0]  GraphicEmissiveColor=[0.0 0.0 0.0 1.0]  GraphicShininess=75  DoExposeReferenceFrame=on  SerializedFrames=<Frames/>
  VisualOriginTransform : sm_lib/Frames and Transforms/Rigid Transform  RotationMethod=RotationSequence  FollAlignAxisA=+X  BaseAlignAxisA=+Y  FollAlignAxisB=+Y  BaseAlignAxisB=+Z  RotationStandardAxis=+Z  RotationAngle=0  RotationAngleUnits=deg  RotationArbitraryAxis=[0 0 1]  RotationSequenceAxes=BaseAxes  RotationSequence=XYZ  RotationSequenceAngles=[0, 0, 0]  RotationSequenceAnglesUnits=rad  RotationMatrix=[1 0 0;0 1 0;0 0 1]  Quaternion=[1 0 0 0]  TranslationMethod=Cartesian  TranslationCartesianOffset=[0, 0, 0]  TranslationCartesianOffsetUnits=m  TranslationStandardAxis=+Z  TranslationStandardOffset=0  TranslationStandardOffsetUnits=m  TranslationROffset=0  TranslationROffsetUnits=m  TranslationThetaOffset=0  TranslationThetaOffsetUnits=deg  TranslationZOffset=0  TranslationZOffsetUnits=m
  F : PMIOPort  Side=Left
  F1 : PMIOPort  Port=2  Side=Right
  connections:
  Visual/RConn1 -- VisualOriginTransform/RConn1
  F/RConn1 -- VisualOriginTransform/LConn1 -- ReferenceFrame/RConn1 -- InertiaOriginTransform/LConn1 -- Joint_1_OriginTransform/LConn1
  Joint_1_AxisTransform/LConn1 -- Joint_1_OriginTransform/RConn1
  Joint_1_AxisTransform/RConn1 -- F1/RConn1
  Inertia/RConn1 -- InertiaOriginTransform/RConn1

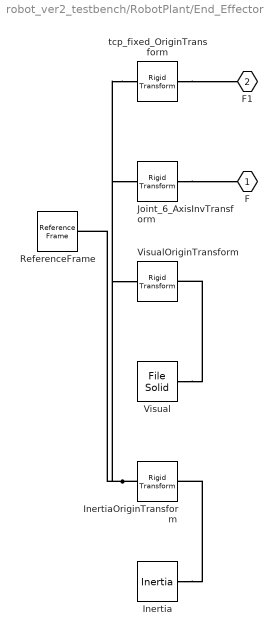
== system robot_ver2_testbench/RobotPlant/End_Effector ==
  Inertia : sm_lib/Body Elements/Inertia  InertiaType=Custom  Mass=1.134  MassUnits=kg  CenterOfMass=[0, 0, 0]  CenterOfMassUnits=m  MomentsOfInertia=[0.005579273, 0.004477524, 0.001211861]  MomentsOfInertiaUnits=kg*m^2  ProductsOfInertia=[0.000351426, 0.000223269, 3.3235e-05]  ProductsOfInertiaUnits=kg*m^2  GraphicType=None  MarkerShape=Inertia  MarkerSize=20  GraphicVisPropType=SimpleVisualProperties  GraphicDiffuseColor=[0.5 0.5 0.5]  GraphicOpacity=1  GraphicSpecularColor=[0.5 0.5 0.5 1.0]  GraphicAmbientColor=[0.15 0.15 0.15 1.0]  GraphicEmissiveColor=[0.0 0.0 0.0 1.0]  GraphicShininess=75
  InertiaOriginTransform : sm_lib/Frames and Transforms/Rigid Transform  RotationMethod=RotationSequence  FollAlignAxisA=+X  BaseAlignAxisA=+Y  FollAlignAxisB=+Y  BaseAlignAxisB=+Z  RotationStandardAxis=+Z  RotationAngle=0  RotationAngleUnits=deg  RotationArbitraryAxis=[0 0 1]  RotationSequenceAxes=BaseAxes  RotationSequence=XYZ  RotationSequenceAngles=[0, 0, 0]  RotationSequenceAnglesUnits=rad  RotationMatrix=[1 0 0;0 1 0;0 0 1]  Quaternion=[1 0 0 0]  TranslationMethod=Cartesian  TranslationCartesianOffset=[-0.008408756, -0.050761756, 0.06633125600000001]  TranslationCartesianOffsetUnits=m  TranslationStandardAxis=+Z  TranslationStandardOffset=0  TranslationStandardOffsetUnits=m  TranslationROffset=0  TranslationROffsetUnits=m  TranslationThetaOffset=0  TranslationThetaOffsetUnits=deg  TranslationZOffset=0  TranslationZOffsetUnits=m
  Joint_6_AxisInvTransform : sm_lib/Frames and Transforms/Rigid Transform  RotationMethod=ArbitraryAxis  FollAlignAxisA=+X  BaseAlignAxisA=+Y  FollAlignAxisB=+Y  BaseAlignAxisB=+Z  RotationStandardAxis=+Z  RotationAngle=0  RotationAngleUnits=rad  RotationArbitraryAxis=[1, 0, 0]  RotationSequenceAxes=FollowerAxes  RotationSequence=XYX  RotationSequenceAngles=[0 0 0]  RotationSequenceAnglesUnits=deg  RotationMatrix=[1 0 0;0 1 0;0 0 1]  Quaternion=[1 0 0 0]  TranslationMethod=Cartesian  TranslationCartesianOffset=[0, 0, 0]  TranslationCartesianOffsetUnits=m  TranslationStandardAxis=+Z  TranslationStandardOffset=0  TranslationStandardOffsetUnits=m  TranslationROffset=0  TranslationROffsetUnits=m  TranslationThetaOffset=0  TranslationThetaOffsetUnits=deg  TranslationZOffset=0  TranslationZOffsetUnits=m
  ReferenceFrame : sm_lib/Frames and Transforms/Reference Frame
  Visual : sm_lib/Body Elements/File Solid  ExtGeomFileName=robot_ver2_End_Effector.STL  UnitType=Custom  ExtGeomFileUnits=m  StepReaderType=HEX  ExportConvexHullGeometry=off  InertiaType=Custom  BasedOnType=DensityFromFile  Density=1000  DensityUnits=kg/m^3  Mass=0  MassUnits=kg  CenterOfMass=[0, 0, 0]  CenterOfMassUnits=m  MomentsOfInertia=[0, 0, 0]  MomentsOfInertiaUnits=kg*m^2  ProductsOfInertia=[0, 0, 0]  ProductsOfInertiaUnits=kg*m^2  GraphicType=FromGeometry  MarkerShape=Sphere  MarkerSize=10  GraphicVisPropType=SimpleVisualProperties  GraphicDiffuseColor=[0.79216, 0.8196099999999999, 0.93333]  GraphicOpacity=1  GraphicSpecularColor=[0.5 0.5 0.5 1.0]  GraphicAmbientColor=[0.15 0.15 0.15 1.0]  GraphicEmissiveColor=[0.0 0.0 0.0 1.0]  GraphicShininess=75  DoExposeReferenceFrame=on  SerializedFrames=<Frames/>
  VisualOriginTransform : sm_lib/Frames and Transforms/Rigid Transform  RotationMethod=RotationSequence  FollAlignAxisA=+X  BaseAlignAxisA=+Y  FollAlignAxisB=+Y  BaseAlignAxisB=+Z  RotationStandardAxis=+Z  RotationAngle=0  RotationAngleUnits=deg  RotationArbitraryAxis=[0 0 1]  RotationSequenceAxes=BaseAxes  RotationSequence=XYZ  RotationSequenceAngles=[0, 0, 0]  RotationSequenceAnglesUnits=rad  RotationMatrix=[1 0 0;0 1 0;0 0 1]  Quaternion=[1 0 0 0]  TranslationMethod=Cartesian  TranslationCartesianOffset=[0, 0, 0]  TranslationCartesianOffsetUnits=m  TranslationStandardAxis=+Z  TranslationStandardOffset=0  TranslationStandardOffsetUnits=m  TranslationROffset=0  TranslationROffsetUnits=m  TranslationThetaOffset=0  TranslationThetaOffsetUnits=deg  TranslationZOffset=0  TranslationZOffsetUnits=m
  tcp_fixed_OriginTransform : sm_lib/Frames and Transforms/Rigid Transform  RotationMethod=RotationSequence  FollAlignAxisA=+X  BaseAlignAxisA=+Y  FollAlignAxisB=+Y  BaseAlignAxisB=+Z  RotationStandardAxis=+Z  RotationAngle=0  RotationAngleUnits=deg  RotationArbitraryAxis=[0 0 1]  RotationSequenceAxes=BaseAxes  RotationSequence=XYZ  RotationSequenceAngles=[0, 0, 0]  RotationSequenceAnglesUnits=rad  RotationMatrix=[1 0 0;0 1 0;0 0 1]  Quaternion=[1 0 0 0]  TranslationMethod=Cartesian  TranslationCartesianOffset=[-0.02287, 0.02053, 0.24577]  TranslationCartesianOffsetUnits=m  TranslationStandardAxis=+Z  TranslationStandardOffset=0  TranslationStandardOffsetUnits=m  TranslationROffset=0  TranslationROffsetUnits=m  TranslationThetaOffset=0  TranslationThetaOffsetUnits=deg  TranslationZOffset=0  TranslationZOffsetUnits=m
  F : PMIOPort  Side=Left
  F1 : PMIOPort  Port=2  Side=Right
  connections:
  tcp_fixed_OriginTransform/RConn1 -- F1/RConn1
  Visual/RConn1 -- VisualOriginTransform/RConn1
  tcp_fixed_OriginTransform/LConn1 -- VisualOriginTransform/LConn1 -- ReferenceFrame/RConn1 -- InertiaOriginTransform/LConn1 -- Joint_6_AxisInvTransform/LConn1
  Joint_6_AxisInvTransform/RConn1 -- F/RConn1
  Inertia/RConn1 -- InertiaOriginTransform/RConn1

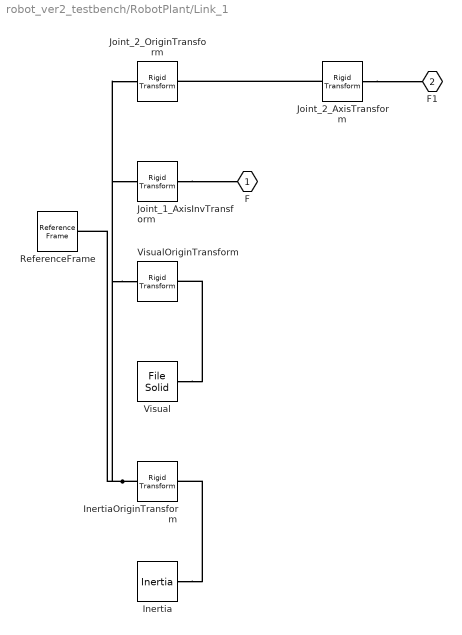
== system robot_ver2_testbench/RobotPlant/Link_1 ==
  Inertia : sm_lib/Body Elements/Inertia  InertiaType=Custom  Mass=4.393  MassUnits=kg  CenterOfMass=[0, 0, 0]  CenterOfMassUnits=m  MomentsOfInertia=[0.017894845, 0.015147419, 0.01203164]  MomentsOfInertiaUnits=kg*m^2  ProductsOfInertia=[0.001949386, 9.7e-07, -1.148e-06]  ProductsOfInertiaUnits=kg*m^2  GraphicType=None  MarkerShape=Inertia  MarkerSize=20  GraphicVisPropType=SimpleVisualProperties  GraphicDiffuseColor=[0.5 0.5 0.5]  GraphicOpacity=1  GraphicSpecularColor=[0.5 0.5 0.5 1.0]  GraphicAmbientColor=[0.15 0.15 0.15 1.0]  GraphicEmissiveColor=[0.0 0.0 0.0 1.0]  GraphicShininess=75
  InertiaOriginTransform : sm_lib/Frames and Transforms/Rigid Transform  RotationMethod=RotationSequence  FollAlignAxisA=+X  BaseAlignAxisA=+Y  FollAlignAxisB=+Y  BaseAlignAxisB=+Z  RotationStandardAxis=+Z  RotationAngle=0  RotationAngleUnits=deg  RotationArbitraryAxis=[0 0 1]  RotationSequenceAxes=BaseAxes  RotationSequence=XYZ  RotationSequenceAngles=[0, 0, 0]  RotationSequenceAnglesUnits=rad  RotationMatrix=[1 0 0;0 1 0;0 0 1]  Quaternion=[1 0 0 0]  TranslationMethod=Cartesian  TranslationCartesianOffset=[-1e-05, -0.024003, 0.114143]  TranslationCartesianOffsetUnits=m  TranslationStandardAxis=+Z  TranslationStandardOffset=0  TranslationStandardOffsetUnits=m  TranslationROffset=0  TranslationROffsetUnits=m  TranslationThetaOffset=0  TranslationThetaOffsetUnits=deg  TranslationZOffset=0  TranslationZOffsetUnits=m
  Joint_1_AxisInvTransform : sm_lib/Frames and Transforms/Rigid Transform  RotationMethod=ArbitraryAxis  FollAlignAxisA=+X  BaseAlignAxisA=+Y  FollAlignAxisB=+Y  BaseAlignAxisB=+Z  RotationStandardAxis=+Z  RotationAngle=3.141592653589793  RotationAngleUnits=rad  RotationArbitraryAxis=[1, 0, 0]  RotationSequenceAxes=FollowerAxes  RotationSequence=XYX  RotationSequenceAngles=[0 0 0]  RotationSequenceAnglesUnits=deg  RotationMatrix=[1 0 0;0 1 0;0 0 1]  Quaternion=[1 0 0 0]  TranslationMethod=Cartesian  TranslationCartesianOffset=[0, 0, 0]  TranslationCartesianOffsetUnits=m  TranslationStandardAxis=+Z  TranslationStandardOffset=0  TranslationStandardOffsetUnits=m  TranslationROffset=0  TranslationROffsetUnits=m  TranslationThetaOffset=0  TranslationThetaOffsetUnits=deg  TranslationZOffset=0  TranslationZOffsetUnits=m
  Joint_2_AxisTransform : sm_lib/Frames and Transforms/Rigid Transform  RotationMethod=ArbitraryAxis  FollAlignAxisA=+X  BaseAlignAxisA=+Y  FollAlignAxisB=+Y  BaseAlignAxisB=+Z  RotationStandardAxis=+Z  RotationAngle=3.141592653589793  RotationAngleUnits=rad  RotationArbitraryAxis=[1, 0, 0]  RotationSequenceAxes=FollowerAxes  RotationSequence=XYX  RotationSequenceAngles=[0 0 0]  RotationSequenceAnglesUnits=deg  RotationMatrix=[1 0 0;0 1 0;0 0 1]  Quaternion=[1 0 0 0]  TranslationMethod=Cartesian  TranslationCartesianOffset=[0, 0, 0]  TranslationCartesianOffsetUnits=m  TranslationStandardAxis=+Z  TranslationStandardOffset=0  TranslationStandardOffsetUnits=m  TranslationROffset=0  TranslationROffsetUnits=m  TranslationThetaOffset=0  TranslationThetaOffsetUnits=deg  TranslationZOffset=0  TranslationZOffsetUnits=m
  Joint_2_OriginTransform : sm_lib/Frames and Transforms/Rigid Transform  RotationMethod=RotationSequence  FollAlignAxisA=+X  BaseAlignAxisA=+Y  FollAlignAxisB=+Y  BaseAlignAxisB=+Z  RotationStandardAxis=+Z  RotationAngle=0  RotationAngleUnits=deg  RotationArbitraryAxis=[0 0 1]  RotationSequenceAxes=BaseAxes  RotationSequence=XYZ  RotationSequenceAngles=[-1.5707963267949, 0, 0]  RotationSequenceAnglesUnits=rad  RotationMatrix=[1 0 0;0 1 0;0 0 1]  Quaternion=[1 0 0 0]  TranslationMethod=Cartesian  TranslationCartesianOffset=[0, -0.08050000000000079, 0.132]  TranslationCartesianOffsetUnits=m  TranslationStandardAxis=+Z  TranslationStandardOffset=0  TranslationStandardOffsetUnits=m  TranslationROffset=0  TranslationROffsetUnits=m  TranslationThetaOffset=0  TranslationThetaOffsetUnits=deg  TranslationZOffset=0  TranslationZOffsetUnits=m
  ReferenceFrame : sm_lib/Frames and Transforms/Reference Frame
  Visual : sm_lib/Body Elements/File Solid  ExtGeomFileName=robot_ver2_Link_1.STL  UnitType=Custom  ExtGeomFileUnits=m  StepReaderType=HEX  ExportConvexHullGeometry=off  InertiaType=Custom  BasedOnType=DensityFromFile  Density=1000  DensityUnits=kg/m^3  Mass=0  MassUnits=kg  CenterOfMass=[0, 0, 0]  CenterOfMassUnits=m  MomentsOfInertia=[0, 0, 0]  MomentsOfInertiaUnits=kg*m^2  ProductsOfInertia=[0, 0, 0]  ProductsOfInertiaUnits=kg*m^2  GraphicType=FromGeometry  MarkerShape=Sphere  MarkerSize=10  GraphicVisPropType=SimpleVisualProperties  GraphicDiffuseColor=[0.792156862745098, 0.819607843137255, 0.933333333333333]  GraphicOpacity=1  GraphicSpecularColor=[0.5 0.5 0.5 1.0]  GraphicAmbientColor=[0.15 0.15 0.15 1.0]  GraphicEmissiveColor=[0.0 0.0 0.0 1.0]  GraphicShininess=75  DoExposeReferenceFrame=on  SerializedFrames=<Frames/>
  VisualOriginTransform : sm_lib/Frames and Transforms/Rigid Transform  RotationMethod=RotationSequence  FollAlignAxisA=+X  BaseAlignAxisA=+Y  FollAlignAxisB=+Y  BaseAlignAxisB=+Z  RotationStandardAxis=+Z  RotationAngle=0  RotationAngleUnits=deg  RotationArbitraryAxis=[0 0 1]  RotationSequenceAxes=BaseAxes  RotationSequence=XYZ  RotationSequenceAngles=[0, 0, 0]  RotationSequenceAnglesUnits=rad  RotationMatrix=[1 0 0;0 1 0;0 0 1]  Quaternion=[1 0 0 0]  TranslationMethod=Cartesian  TranslationCartesianOffset=[0, 0, 0]  TranslationCartesianOffsetUnits=m  TranslationStandardAxis=+Z  TranslationStandardOffset=0  TranslationStandardOffsetUnits=m  TranslationROffset=0  TranslationROffsetUnits=m  TranslationThetaOffset=0  TranslationThetaOffsetUnits=deg  TranslationZOffset=0  TranslationZOffsetUnits=m
  F : PMIOPort  Side=Left
  F1 : PMIOPort  Port=2  Side=Right
  connections:
  Visual/RConn1 -- VisualOriginTransform/RConn1
  VisualOriginTransform/LConn1 -- ReferenceFrame/RConn1 -- Joint_2_OriginTransform/LConn1 -- InertiaOriginTransform/LConn1 -- Joint_1_AxisInvTransform/LConn1
  Joint_2_AxisTransform/LConn1 -- Joint_2_OriginTransform/RConn1
  Joint_2_AxisTransform/RConn1 -- F1/RConn1
  Joint_1_AxisInvTransform/RConn1 -- F/RConn1
  Inertia/RConn1 -- InertiaOriginTransform/RConn1

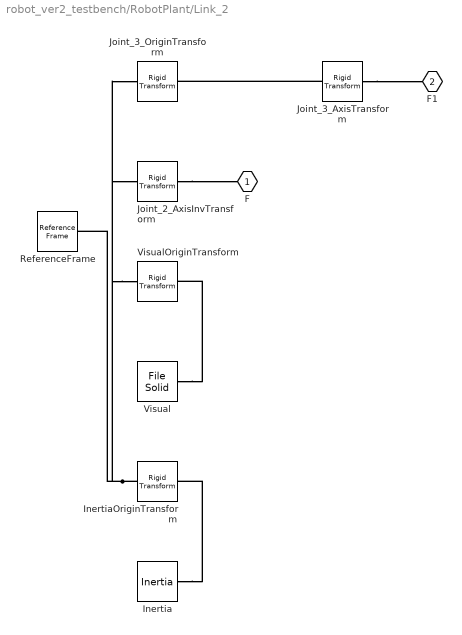
== system robot_ver2_testbench/RobotPlant/Link_2 ==
  Inertia : sm_lib/Body Elements/Inertia  InertiaType=Custom  Mass=5.113  MassUnits=kg  CenterOfMass=[0, 0, 0]  CenterOfMassUnits=m  MomentsOfInertia=[0.235463496, 0.030331894, 0.221411808]  MomentsOfInertiaUnits=kg*m^2  ProductsOfInertia=[-0.034873247, 0, -3e-09]  ProductsOfInertiaUnits=kg*m^2  GraphicType=None  MarkerShape=Inertia  MarkerSize=20  GraphicVisPropType=SimpleVisualProperties  GraphicDiffuseColor=[0.5 0.5 0.5]  GraphicOpacity=1  GraphicSpecularColor=[0.5 0.5 0.5 1.0]  GraphicAmbientColor=[0.15 0.15 0.15 1.0]  GraphicEmissiveColor=[0.0 0.0 0.0 1.0]  GraphicShininess=75
  InertiaOriginTransform : sm_lib/Frames and Transforms/Rigid Transform  RotationMethod=RotationSequence  FollAlignAxisA=+X  BaseAlignAxisA=+Y  FollAlignAxisB=+Y  BaseAlignAxisB=+Z  RotationStandardAxis=+Z  RotationAngle=0  RotationAngleUnits=deg  RotationArbitraryAxis=[0 0 1]  RotationSequenceAxes=BaseAxes  RotationSequence=XYZ  RotationSequenceAngles=[0, 0, 0]  RotationSequenceAnglesUnits=rad  RotationMatrix=[1 0 0;0 1 0;0 0 1]  Quaternion=[1 0 0 0]  TranslationMethod=Cartesian  TranslationCartesianOffset=[0, -0.295232, -0.186319]  TranslationCartesianOffsetUnits=m  TranslationStandardAxis=+Z  TranslationStandardOffset=0  TranslationStandardOffsetUnits=m  TranslationROffset=0  TranslationROffsetUnits=m  TranslationThetaOffset=0  TranslationThetaOffsetUnits=deg  TranslationZOffset=0  TranslationZOffsetUnits=m
  Joint_2_AxisInvTransform : sm_lib/Frames and Transforms/Rigid Transform  RotationMethod=ArbitraryAxis  FollAlignAxisA=+X  BaseAlignAxisA=+Y  FollAlignAxisB=+Y  BaseAlignAxisB=+Z  RotationStandardAxis=+Z  RotationAngle=3.141592653589793  RotationAngleUnits=rad  RotationArbitraryAxis=[1, 0, 0]  RotationSequenceAxes=FollowerAxes  RotationSequence=XYX  RotationSequenceAngles=[0 0 0]  RotationSequenceAnglesUnits=deg  RotationMatrix=[1 0 0;0 1 0;0 0 1]  Quaternion=[1 0 0 0]  TranslationMethod=Cartesian  TranslationCartesianOffset=[0, 0, 0]  TranslationCartesianOffsetUnits=m  TranslationStandardAxis=+Z  TranslationStandardOffset=0  TranslationStandardOffsetUnits=m  TranslationROffset=0  TranslationROffsetUnits=m  TranslationThetaOffset=0  TranslationThetaOffsetUnits=deg  TranslationZOffset=0  TranslationZOffsetUnits=m
  Joint_3_AxisTransform : sm_lib/Frames and Transforms/Rigid Transform  RotationMethod=ArbitraryAxis  FollAlignAxisA=+X  BaseAlignAxisA=+Y  FollAlignAxisB=+Y  BaseAlignAxisB=+Z  RotationStandardAxis=+Z  RotationAngle=0  RotationAngleUnits=rad  RotationArbitraryAxis=[1, 0, 0]  RotationSequenceAxes=FollowerAxes  RotationSequence=XYX  RotationSequenceAngles=[0 0 0]  RotationSequenceAnglesUnits=deg  RotationMatrix=[1 0 0;0 1 0;0 0 1]  Quaternion=[1 0 0 0]  TranslationMethod=Cartesian  TranslationCartesianOffset=[0, 0, 0]  TranslationCartesianOffsetUnits=m  TranslationStandardAxis=+Z  TranslationStandardOffset=0  TranslationStandardOffsetUnits=m  TranslationROffset=0  TranslationROffsetUnits=m  TranslationThetaOffset=0  TranslationThetaOffsetUnits=deg  TranslationZOffset=0  TranslationZOffsetUnits=m
  Joint_3_OriginTransform : sm_lib/Frames and Transforms/Rigid Transform  RotationMethod=RotationSequence  FollAlignAxisA=+X  BaseAlignAxisA=+Y  FollAlignAxisB=+Y  BaseAlignAxisB=+Z  RotationStandardAxis=+Z  RotationAngle=0  RotationAngleUnits=deg  RotationArbitraryAxis=[0 0 1]  RotationSequenceAxes=BaseAxes  RotationSequence=XYZ  RotationSequenceAngles=[0, 0, 0]  RotationSequenceAnglesUnits=rad  RotationMatrix=[1 0 0;0 1 0;0 0 1]  Quaternion=[1 0 0 0]  TranslationMethod=Cartesian  TranslationCartesianOffset=[0, -0.589954679438418, -0.155500000000012]  TranslationCartesianOffsetUnits=m  TranslationStandardAxis=+Z  TranslationStandardOffset=0  TranslationStandardOffsetUnits=m  TranslationROffset=0  TranslationROffsetUnits=m  TranslationThetaOffset=0  TranslationThetaOffsetUnits=deg  TranslationZOffset=0  TranslationZOffsetUnits=m
  ReferenceFrame : sm_lib/Frames and Transforms/Reference Frame
  Visual : sm_lib/Body Elements/File Solid  ExtGeomFileName=robot_ver2_Link_2.STL  UnitType=Custom  ExtGeomFileUnits=m  StepReaderType=HEX  ExportConvexHullGeometry=off  InertiaType=Custom  BasedOnType=DensityFromFile  Density=1000  DensityUnits=kg/m^3  Mass=0  MassUnits=kg  CenterOfMass=[0, 0, 0]  CenterOfMassUnits=m  MomentsOfInertia=[0, 0, 0]  MomentsOfInertiaUnits=kg*m^2  ProductsOfInertia=[0, 0, 0]  ProductsOfInertiaUnits=kg*m^2  GraphicType=FromGeometry  MarkerShape=Sphere  MarkerSize=10  GraphicVisPropType=SimpleVisualProperties  GraphicDiffuseColor=[0.792156862745098, 0.819607843137255, 0.933333333333333]  GraphicOpacity=1  GraphicSpecularColor=[0.5 0.5 0.5 1.0]  GraphicAmbientColor=[0.15 0.15 0.15 1.0]  GraphicEmissiveColor=[0.0 0.0 0.0 1.0]  GraphicShininess=75  DoExposeReferenceFrame=on  SerializedFrames=<Frames/>
  VisualOriginTransform : sm_lib/Frames and Transforms/Rigid Transform  RotationMethod=RotationSequence  FollAlignAxisA=+X  BaseAlignAxisA=+Y  FollAlignAxisB=+Y  BaseAlignAxisB=+Z  RotationStandardAxis=+Z  RotationAngle=0  RotationAngleUnits=deg  RotationArbitraryAxis=[0 0 1]  RotationSequenceAxes=BaseAxes  RotationSequence=XYZ  RotationSequenceAngles=[0, 0, 0]  RotationSequenceAnglesUnits=rad  RotationMatrix=[1 0 0;0 1 0;0 0 1]  Quaternion=[1 0 0 0]  TranslationMethod=Cartesian  TranslationCartesianOffset=[0, 0, 0]  TranslationCartesianOffsetUnits=m  TranslationStandardAxis=+Z  TranslationStandardOffset=0  TranslationStandardOffsetUnits=m  TranslationROffset=0  TranslationROffsetUnits=m  TranslationThetaOffset=0  TranslationThetaOffsetUnits=deg  TranslationZOffset=0  TranslationZOffsetUnits=m
  F : PMIOPort  Side=Left
  F1 : PMIOPort  Port=2  Side=Right
  connections:
  Visual/RConn1 -- VisualOriginTransform/RConn1
  VisualOriginTransform/LConn1 -- ReferenceFrame/RConn1 -- Joint_3_OriginTransform/LConn1 -- InertiaOriginTransform/LConn1 -- Joint_2_AxisInvTransform/LConn1
  Joint_3_AxisTransform/LConn1 -- Joint_3_OriginTransform/RConn1
  Joint_3_AxisTransform/RConn1 -- F1/RConn1
  Joint_2_AxisInvTransform/RConn1 -- F/RConn1
  Inertia/RConn1 -- InertiaOriginTransform/RConn1
